simulink model "a"  (R2022b)
settings: Solver=VariableStepAuto  StartTime=0.0  StopTime=10.0  RelTol=1e-3
settings Model: Creator=260910-7  LastModifiedBy=260910-7

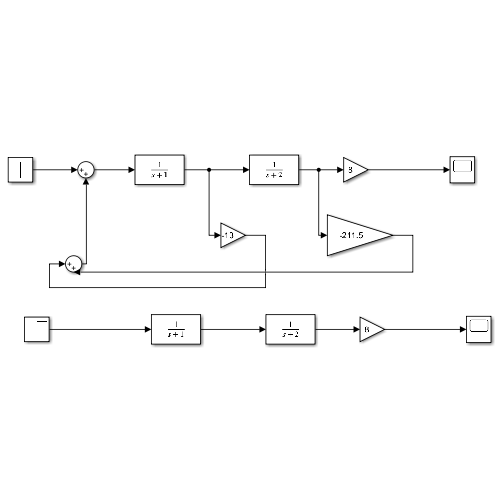
[thumbnail: Simulink's stored preview of the top-level diagram]
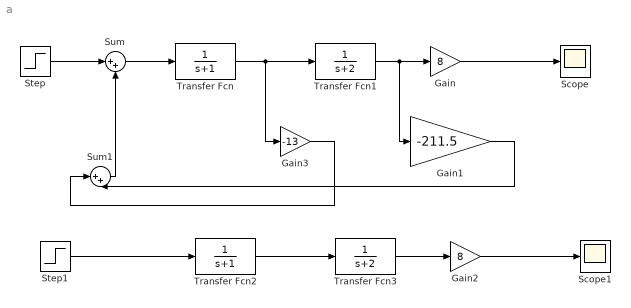
== system a ==
  Gain : Gain  Gain=8
  Gain1 : Gain  Gain=-211.5
  Gain2 : Gain  Gain=8
  Gain3 : Gain  Gain=-13
  Scope : Scope
  Scope1 : Scope
  Step : Step  Time=0  After=4  SampleTime=0
  Step1 : Step  Time=0  After=4  SampleTime=0
  Sum : Sum  Inputs=|++
  Sum1 : Sum  Inputs=|++
  Transfer Fcn : TransferFcn  Denominator=[1 1]
  Transfer Fcn1 : TransferFcn  Denominator=[1 2]
  Transfer Fcn2 : TransferFcn  Denominator=[1 1]
  Transfer Fcn3 : TransferFcn  Denominator=[1 2]
  wires:
  Transfer Fcn/1 -> Gain3/1, Transfer Fcn1/1
  Transfer Fcn1/1 -> Gain1/1, Gain/1
  Gain/1 -> Scope/1
  Gain1/1 -> Sum1/2
  Gain3/1 -> Sum1/1
  Step/1 -> Sum/1
  Sum/1 -> Transfer Fcn/1
  Sum1/1 -> Sum/2
  Transfer Fcn2/1 -> Transfer Fcn3/1
  Gain2/1 -> Scope1/1
  Transfer Fcn3/1 -> Gain2/1
  Step1/1 -> Transfer Fcn2/1
